simulink model "vishva_4"  (R2018b)
settings: Solver=VariableStepDiscrete  StartTime=0.0  StopTime=10.0  RelTol=1e-3
libraries: powerlib x4, simulink x2
settings Model: Creator=Admin  LastModifiedBy=Admin

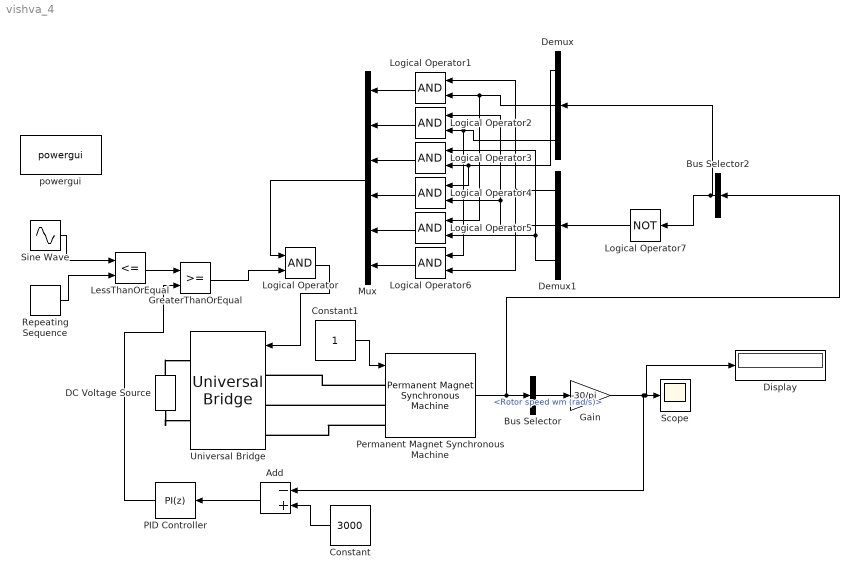
== system vishva_4 ==
  Add : Sum  Inputs=-+
  Bus Selector : BusSelector  OutputSignals=Rotor speed wm (rad/s)
  Bus Selector2 : BusSelector  OutputSignals=Hall effect signal h_a,Hall effect signal h_b,Hall effect signal h_c  OutputAsBus=on
  Constant : Constant  Value=3000  SampleTime=-1
  Constant1 : Constant  VectorParams1D=off  SampleTime=-1
  DC Voltage Source : powerlib/Electrical Sources/DC Voltage Source  Amplitude=400  Measurements=Voltage
  Demux : Demux  Outputs=3
  Demux1 : Demux  Outputs=3
  Display : Display
  Gain : Gain  Gain=-30/pi
  GreaterThanOrEqual : RelationalOperator  OutDataTypeStr=boolean  RndMeth=Simplest
  LessThanOrEqual : RelationalOperator  Operator=<=  OutDataTypeStr=boolean  RndMeth=Simplest
  Logical Operator{,1..6} (7 alike) : Logic  AllPortsSameDT=off  OutDataTypeStr=boolean
  Logical Operator7 : Logic  Operator=NOT  AllPortsSameDT=off  OutDataTypeStr=boolean
  Mux : Mux  Inputs=6
  PID Controller : simulink/Continuous/PID Controller  Controller=PI  Form=Parallel  TimeDomain=Discrete-time  SampleTime=-1  IntegratorMethod=Forward Euler  FilterMethod=Forward Euler  ControllerParametersSource=internal  P=1  I=10  D=0  UseFilter=on  N=100  TunerSelectOption=Transfer Function Based (PID Tuner App)  ZeroCross=off  InitialConditionSource=internal  InitialConditionForIntegrator=0  InitialConditionForFilter=0  DifferentiatorICPrevScaledInput=0  ExternalReset=none  TrackingMode=off  Kt=1  LimitOutput=off  UpperSaturationLimit=inf  LowerSaturationLimit=-inf  LinearizeAsGain=on  AntiWindupMode=none  Kb=1  POutMin=[]  POutMax=[]  IOutMin=[]  IOutMax=[]  DOutMin=[]  DOutMax=[]  NOutMin=[]  NOutMax=[]  SumOutMin=[]  SumOutMax=[]  SaturationOutMin=[]  SaturationOutMax=[]  PParamMin=[]  PParamMax=[]  IParamMin=[]  IParamMax=[]  DParamMin=[]  DParamMax=[]  NParamMin=[]  NParamMax=[]  KbParamMin=[]  KbParamMax=[]  KtParamMin=[]  KtParamMax=[]  KbOutMin=[]  KbOutMax=[]  KtOutMin=[]  KtOutMax=[]  IntegratorOutMin=[]  IntegratorOutMax=[]  FilterOutMin=[]  FilterOutMax=[]  SumI1OutMin=[]  SumI1OutMax=[]  SumI2OutMin=[]  SumI2OutMax=[]  SumI3OutMin=[]  SumI3OutMax=[]  SumI4OutMin=[]  SumI4OutMax=[]  SumDOutMin=[]  SumDOutMax=[]  DifferentiatorOutMin=[]  DifferentiatorOutMax=[]  FilterDiffOutCoefMin=[]  FilterDiffOutCoefMax=[]  ReciprocalOutMin=[]  ReciprocalOutMax=[]  SumDenOutMin=[]  SumDenOutMax=[]  SumNumOutMin=[]  SumNumOutMax=[]  DivideOutMin=[]  DivideOutMax=[]  IntegratorContinuousStateAttributes=''  IntegratorStateMustResolveToSignalObject=off  IntegratorRTWStateStorageClass=Auto  FilterContinuousStateAttributes=''  FilterStateMustResolveToSignalObject=off  FilterRTWStateStorageClass=Auto  ParallelPVariant=InternalParameters  IdealPVariant=Disabled  IVariant=InternalParameters  DVariant=Disabled  IntegratorVariant=Discrete  SatVariant=Disabled  AWVariant=Passthrough  PCopyVariant=Disabled  TRVariant=Disabled  FdbkBlocksVariant=Forward  IdealPFdbkVariant=Disabled  SatFdbkVariant=Disabled  DerivativeFilterVariant=Disabled  NVariant=Disabled  NCopyVariant=Disabled_SignalSpec  FilterICVariant=Disabled  IntegratorICVariant=InternalICs  ExternalResetVariant=Disabled  TRSumVariant=Passthrough  SumFdbkVariant=Disabled  SumVariant=Sum_PI
  Permanent Magnet Synchronous Machine : powerlib/Machines/Permanent Magnet Synchronous Machine  NbPhases=3  FluxDistribution=Trapezoidal  RotorType=Round  MechanicalLoad=Torque Tm  PresetModel=No  ShowDetailedParameters=on  MeasurementBus=off  Resistance=0.0485  Inductance=8.5e-3  dqInductances=[8.5e-3,8.5e-3]  La=0.000395  MachineConstant=Flux linkage established by magnets (V.s)  Flux=0.1194  VoltageCst=100.0283  TorqueCst=0.9552  Flat=120  Mechanical=[0.0027 0.0004924 4 0]  PolePairs=4  InitialConditions=[0,0, 0,0]  InitialConditions5ph=[0 0 0 0 0 0]  TsPowergui=0  TsBlock=-1  RefAngle=90 degrees behind phase A axis (modified Park)
      settings: SourceProductName=Simscape Power Systems
  Repeating Sequence : simulink/Sources/Repeating Sequence  rep_seq_t=[0 2]  rep_seq_y=[0 2]
  Scope : Scope
  Sine Wave : Sin  SampleTime=0
  Universal Bridge : powerlib/Power Electronics/Universal Bridge  Arms=3  SnubberResistance=1e5  SnubberCapacitance=inf  Device=MOSFET / Diodes  Ron=1e-3  Lon=0  ForwardVoltages="[  0  0  ]"  ForwardVoltage=0  GTOparameters=[ 10e-6 , 20e-6 ]  IGBTparameters=[ 1e-6 , 2e-6 ]  Measurements=None  Measurements_2=None  converterType=Rectifier
  powergui : powerlib/powergui  Priority=1  SimulationMode=Discrete  SampleTime=5e-05  frequency=60  Iterations=50  frequencyindice=0  Pbase=100e6  ErrMax=1e-4  UnitsV=kV  UnitsW=MW  buscounter=0  FunctionMessages=off  echomessages=off  EnableUseOfTLC=off  CurrentSourceSwitches=off  DisableSnubberDevices=off  DisableRonSwitches=off  DisableVfSwitches=off  DisplayEquations=off  SolverType=Tustin/Backward Euler (TBE)  Interpol=off  ExternalGateDelay=off  methode=off  Ts=100  x0status=blocks  SPID=on  SwTol=0  HookPort=off  RestoreLinks=warning  ResistiveCurrentMeasurement=off  Frange=[0:2:500]  Ylog=off  Xlog=on  ShowGrid=off  save=off  variable=ZData  structure=0  ZoomFFT=off  StartTime=0.0  cycles=1  DisplayStyle=1  fundamental=60  FreqAxis=off  MaxFrequency=1000  frequencyindicesteady=1  RmsSteady=1  display=off
  wires:
  Logical Operator1/1 -> Mux/1
  Logical Operator2/1 -> Mux/2
  Logical Operator3/1 -> Mux/3
  Logical Operator4/1 -> Mux/4
  Logical Operator5/1 -> Mux/5
  Logical Operator6/1 -> Mux/6
  Constant/1 -> Add/2
  Add/1 -> PID Controller/1
  Sine Wave/1 -> LessThanOrEqual/1
  Repeating Sequence/1 -> LessThanOrEqual/2
  LessThanOrEqual/1 -> GreaterThanOrEqual/1
  Constant1/1 -> Permanent Magnet Synchronous Machine/1
  Permanent Magnet Synchronous Machine/1 -> Bus Selector2/1, Bus Selector/1
  Gain/1 -> Add/1, Display/1, Scope/1
  Bus Selector/1 -> Gain/1  "<Rotor speed wm (rad/s)>"
  Logical Operator7/1 -> Demux1/1
  Bus Selector2/1 -> Demux/1, Logical Operator7/1
  PID Controller/1 -> GreaterThanOrEqual/2
  Logical Operator/1 -> Universal Bridge/1
  GreaterThanOrEqual/1 -> Logical Operator/2
  Mux/1 -> Logical Operator/1
  Demux/2 -> Logical Operator5/1, Logical Operator1/2
  Demux1/2 -> Logical Operator4/2, Logical Operator2/1
  Demux1/1 -> Logical Operator6/2, Logical Operator1/1
  Demux/3 -> Logical Operator6/1, Logical Operator2/2
  Demux1/3 -> Logical Operator5/2, Logical Operator3/1
  Demux/1 -> Logical Operator4/1, Logical Operator3/2
  connections:
  Permanent Magnet Synchronous Machine/LConn1 -- Universal Bridge/LConn1
  Permanent Magnet Synchronous Machine/LConn2 -- Universal Bridge/LConn2
  Permanent Magnet Synchronous Machine/LConn3 -- Universal Bridge/LConn3
  DC Voltage Source/RConn1 -- Universal Bridge/RConn1
  DC Voltage Source/LConn1 -- Universal Bridge/RConn2
